simulink model "PDU"  (R2026b)
settings: Solver=VariableStepAuto
undefined symbols (not defined in the file or in its folder): P, Ts
libraries: nesl_utility x25, ee_lib x17, fl_lib x16, simulink x6, eeGeneralControl x3
settings Model: Creator=aomar  LastModifiedBy=aomar

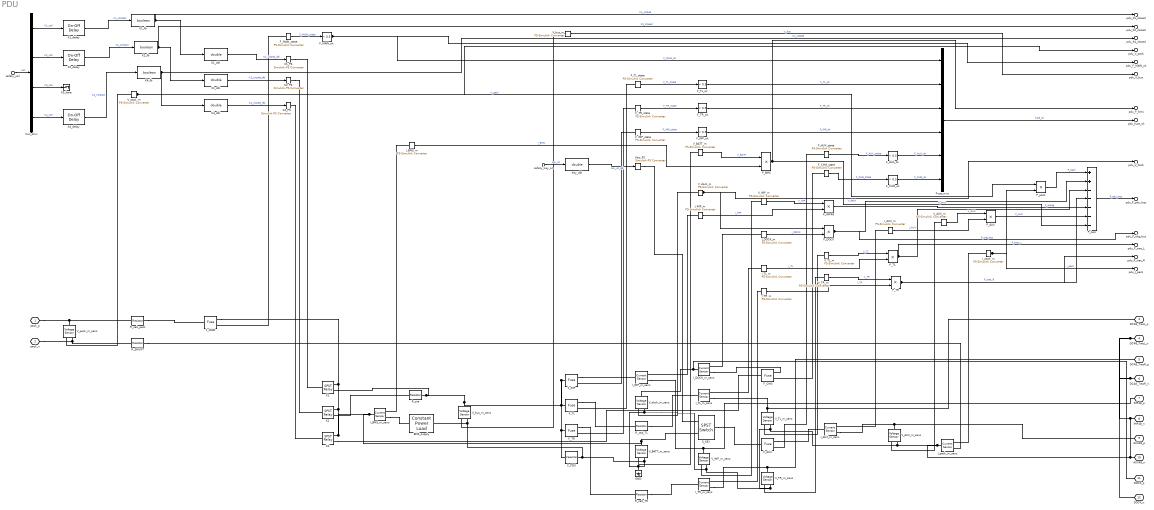
== system PDU ==
  safety_coil : Inport  PortName=safety  Element=coil
  safety_key_on : Inport  PortName=safety  Element=key_on
  BMS_supply : ee_lib/Passive/Constant Power Load  load_type=ee.enum.dc_ac.dc  consumed_power=P.power.pdu.P_bms_supply W  min_supply_voltage=20 V  G_reverse=1e-6 S  deltaV=1e-3 V  active_power=500 W  reactive_power=0 A*V  f0=60 Hz  Vrms_min=200 V  tau=0.01 s  Vrms_ini=300 V  Vang_ini=0 deg
  C_PDU : ee_lib/Passive/Capacitor  cap_option=ee.enum.passive.capacitor.capOption.const  c=P.power.pdu.C_pdu F  Cvec=[1e-05, 1e-06] F  Vvec=[0, 10] V  CV_table_symmetry=ee.enum.passive.capacitor.tableSymmetry.yes  f_vec=[1, 10] kHz  DFext_vec=[.8, 1.2]  enable_C_tol=ee.enum.toleranceApplication.none  averaging_period=0 s  C_tol=5  tol_distribution=ee.enum.toleranceDistribution.uniform  nSigma=4  r=P.power.pdu.ESR_pdu Ohm  g=P.power.pdu.g_bleed 1/Ohm  enable_operating_limits=ee.enum.enable.no  operating_limit_action=ee.enum.passive.reportOpLim.warn  max_working_voltage_range=[-25, 25] V  power_rating=1 W  maxTemperature=85 degC  thermalEnable=false  thermalMass=1 J/K  i_specify=off  i_priority=None  i=0 A  i_nominal_specify=off  i_nominal_value=1  i_nominal_unit=A  v_specify=off  v_priority=None  v=0 V  v_nominal_specify=off  v_nominal_value=1  v_nominal_unit=V  vc_specify=on  vc_priority=High  vc=0 V  vc_nominal_specify=off  vc_nominal_value=1  vc_nominal_unit=V  T_specify=off  T_priority=None  T=298.15 K  T_nominal_specify=off  T_nominal_value=1  T_nominal_unit=K
  Coil_dmx : Demux
  F_AUX : ee_lib/Switches & Breakers/Fuse  prm=3  I_rated=1 A  melt_margin=1  T_fuse=0 s  I2t=1 A^2*s  I_vec=P.power.pdu.F_AUX.I_vec A  t_vec=P.power.pdu.F_AUX.t_vec s  R_closed=P.power.pdu.F_AUX.R_closed Ohm  G_open=P.power.pdu.F_AUX.G_open 1/Ohm  exposemeasurement=ee.enum.exposemeasurement.visible
  F_AUX_ok : simulink/Logic and Bit Operations/Compare To Constant  relop=<  const=0.5  OutDataTypeStr=boolean
  F_AUX_state : nesl_utility/PS-Simulink Converter  PhysicalDomain=network_engine_domain  SubClassName=ps_output  LeftPortType=input  RightPortType=output  PseudoPeriodic=off  Frequencies=[]  VectorFormat=inherit  Unit=1  AffineConversion=off
  F_CHG : ee_lib/Switches & Breakers/Fuse  prm=3  I_rated=1 A  melt_margin=1  T_fuse=0 s  I2t=1 A^2*s  I_vec=P.power.pdu.F_CHG.I_vec A  t_vec=P.power.pdu.F_CHG.t_vec s  R_closed=P.power.pdu.F_CHG.R_closed Ohm  G_open=P.power.pdu.F_CHG.G_open 1/Ohm  exposemeasurement=ee.enum.exposemeasurement.visible
  F_CHG_ok : simulink/Logic and Bit Operations/Compare To Constant  relop=<  const=0.5  OutDataTypeStr=boolean
  F_CHG_state : nesl_utility/PS-Simulink Converter  PhysicalDomain=network_engine_domain  SubClassName=ps_output  LeftPortType=input  RightPortType=output  PseudoPeriodic=off  Frequencies=[]  VectorFormat=inherit  Unit=1  AffineConversion=off
  F_IMP : ee_lib/Switches & Breakers/Fuse  prm=3  I_rated=1 A  melt_margin=1  T_fuse=0 s  I2t=1 A^2*s  I_vec=P.power.pdu.F_IMP.I_vec A  t_vec=P.power.pdu.F_IMP.t_vec s  R_closed=P.power.pdu.F_IMP.R_closed Ohm  G_open=P.power.pdu.F_IMP.G_open 1/Ohm  exposemeasurement=ee.enum.exposemeasurement.visible
  F_IMP_ok : simulink/Logic and Bit Operations/Compare To Constant  relop=<  const=0.5  OutDataTypeStr=boolean
  F_IMP_state : nesl_utility/PS-Simulink Converter  PhysicalDomain=network_engine_domain  SubClassName=ps_output  LeftPortType=input  RightPortType=output  PseudoPeriodic=off  Frequencies=[]  VectorFormat=inherit  Unit=1  AffineConversion=off
  F_MAIN : ee_lib/Switches & Breakers/Fuse  prm=3  I_rated=1 A  melt_margin=1  T_fuse=0 s  I2t=1 A^2*s  I_vec=P.power.pdu.F_MAIN.I_vec A  t_vec=P.power.pdu.F_MAIN.t_vec s  R_closed=P.power.pdu.F_MAIN.R_closed Ohm  G_open=P.power.pdu.F_MAIN.G_open 1/Ohm  exposemeasurement=ee.enum.exposemeasurement.visible
  F_MAIN_ok : simulink/Logic and Bit Operations/Compare To Constant  relop=<  const=0.5  OutDataTypeStr=boolean
  F_MAIN_state : nesl_utility/PS-Simulink Converter  PhysicalDomain=network_engine_domain  SubClassName=ps_output  LeftPortType=input  RightPortType=output  PseudoPeriodic=off  Frequencies=[]  VectorFormat=inherit  Unit=1  AffineConversion=off
  F_TL : ee_lib/Switches & Breakers/Fuse  prm=3  I_rated=1 A  melt_margin=1  T_fuse=0 s  I2t=1 A^2*s  I_vec=P.power.pdu.F_TL.I_vec A  t_vec=P.power.pdu.F_TL.t_vec s  R_closed=P.power.pdu.F_TL.R_closed Ohm  G_open=P.power.pdu.F_TL.G_open 1/Ohm  exposemeasurement=ee.enum.exposemeasurement.visible
  F_TL_ok : simulink/Logic and Bit Operations/Compare To Constant  relop=<  const=0.5  OutDataTypeStr=boolean
  F_TL_state : nesl_utility/PS-Simulink Converter  PhysicalDomain=network_engine_domain  SubClassName=ps_output  LeftPortType=input  RightPortType=output  PseudoPeriodic=off  Frequencies=[]  VectorFormat=inherit  Unit=1  AffineConversion=off
  F_TR : ee_lib/Switches & Breakers/Fuse  prm=3  I_rated=1 A  melt_margin=1  T_fuse=0 s  I2t=1 A^2*s  I_vec=P.power.pdu.F_TR.I_vec A  t_vec=P.power.pdu.F_TR.t_vec s  R_closed=P.power.pdu.F_TR.R_closed Ohm  G_open=P.power.pdu.F_TR.G_open 1/Ohm  exposemeasurement=ee.enum.exposemeasurement.visible
  F_TR_ok : simulink/Logic and Bit Operations/Compare To Constant  relop=<  const=0.5  OutDataTypeStr=boolean
  F_TR_state : nesl_utility/PS-Simulink Converter  PhysicalDomain=network_engine_domain  SubClassName=ps_output  LeftPortType=input  RightPortType=output  PseudoPeriodic=off  Frequencies=[]  VectorFormat=inherit  Unit=1  AffineConversion=off
  Fuse_mux : Mux  Inputs=6
  GND : fl_lib/Electrical/Electrical Elements/Electrical Reference
  I_AUX_m : nesl_utility/PS-Simulink Converter  PhysicalDomain=network_engine_domain  SubClassName=ps_output  LeftPortType=input  RightPortType=output  PseudoPeriodic=off  Frequencies=[]  VectorFormat=inherit  Unit=A  AffineConversion=off
  I_AUX_m_sens : fl_lib/Electrical/Electrical Sensors/Current Sensor
  I_BMS_m : nesl_utility/PS-Simulink Converter  PhysicalDomain=network_engine_domain  SubClassName=ps_output  LeftPortType=input  RightPortType=output  PseudoPeriodic=off  Frequencies=[]  VectorFormat=inherit  Unit=A  AffineConversion=off
  I_BMS_m_sens : fl_lib/Electrical/Electrical Sensors/Current Sensor
  I_DOCK_m : nesl_utility/PS-Simulink Converter  PhysicalDomain=network_engine_domain  SubClassName=ps_output  LeftPortType=input  RightPortType=output  PseudoPeriodic=off  Frequencies=[]  VectorFormat=inherit  Unit=A  AffineConversion=off
  I_DOCK_m_sens : fl_lib/Electrical/Electrical Sensors/Current Sensor
  I_IMP_m : nesl_utility/PS-Simulink Converter  PhysicalDomain=network_engine_domain  SubClassName=ps_output  LeftPortType=input  RightPortType=output  PseudoPeriodic=off  Frequencies=[]  VectorFormat=inherit  Unit=A  AffineConversion=off
  I_IMP_m_sens : fl_lib/Electrical/Electrical Sensors/Current Sensor
  I_TL_m : nesl_utility/PS-Simulink Converter  PhysicalDomain=network_engine_domain  SubClassName=ps_output  LeftPortType=input  RightPortType=output  PseudoPeriodic=off  Frequencies=[]  VectorFormat=inherit  Unit=A  AffineConversion=off
  I_TL_m_sens : fl_lib/Electrical/Electrical Sensors/Current Sensor
  I_TR_m : nesl_utility/PS-Simulink Converter  PhysicalDomain=network_engine_domain  SubClassName=ps_output  LeftPortType=input  RightPortType=output  PseudoPeriodic=off  Frequencies=[]  VectorFormat=inherit  Unit=A  AffineConversion=off
  I_TR_m_sens : fl_lib/Electrical/Electrical Sensors/Current Sensor
  I_pack_m : nesl_utility/PS-Simulink Converter  PhysicalDomain=network_engine_domain  SubClassName=ps_output  LeftPortType=input  RightPortType=output  PseudoPeriodic=off  Frequencies=[]  VectorFormat=inherit  Unit=A  AffineConversion=off
  I_pack_m_sens : fl_lib/Electrical/Electrical Sensors/Current Sensor
  K1 : ee_lib/Switches & Breakers/Relays/SPST Relay  block_choices=ee.enum.controlport.ps  R_closed=P.power.pdu.K1.R_closed Ohm  G_open=P.power.pdu.K1.G_open 1/Ohm  Threshold=0.5  exposemeasurement=ee.enum.exposemeasurement.hidden  V_rated=5 V  V_energize=75  V_deenergize=25  l_winding=0.08 H  r_winding=12.5 Ohm  g_winding=1e-9 1/Ohm  T_brk_C_S=0 s  T_mak_C_S=0 s  fault_types=ee.enum.relays.faultTypes.winding
  K1_PS : nesl_utility/Simulink-PS Converter  PhysicalDomain=network_engine_domain  SubClassName=ps_input  LeftPortType=input  RightPortType=output  PseudoPeriodic=off  Frequencies=[]  NoiseDistribution=none  NoiseParameters=[]  Unit=1  AffineConversion=off  FilteringAndDerivatives=zero  SimscapeFilterOrder=1  InputFilterTimeConstant=0.001  UdotUserProvided=0
  K1_dbl : DataTypeConversion  OutDataTypeStr=double  SaturateOnIntegerOverflow=off  RndMeth=Floor
  K1_delay : eeGeneralControl/On-Off Delay  LabelModeActiveChoice=Discrete  Td_on=P.power.pdu.K1.t_on  Td_off=P.power.pdu.K1.t_off  IC=0  Ts=Ts.base
      settings: LibrarySourceBlock=ee_sl_lib/General Control/On-Off Delay
  K1_fb : DataTypeConversion  OutDataTypeStr=boolean  RndMeth=Nearest
  K2 : ee_lib/Switches & Breakers/Relays/SPST Relay  block_choices=ee.enum.controlport.ps  R_closed=P.power.pdu.K2.R_closed Ohm  G_open=P.power.pdu.K2.G_open 1/Ohm  Threshold=0.5  exposemeasurement=ee.enum.exposemeasurement.hidden  V_rated=5 V  V_energize=75  V_deenergize=25  l_winding=0.08 H  r_winding=12.5 Ohm  g_winding=1e-9 1/Ohm  T_brk_C_S=0 s  T_mak_C_S=0 s  fault_types=ee.enum.relays.faultTypes.winding
  K2_PS : nesl_utility/Simulink-PS Converter  PhysicalDomain=network_engine_domain  SubClassName=ps_input  LeftPortType=input  RightPortType=output  PseudoPeriodic=off  Frequencies=[]  NoiseDistribution=none  NoiseParameters=[]  Unit=1  AffineConversion=off  FilteringAndDerivatives=zero  SimscapeFilterOrder=1  InputFilterTimeConstant=0.001  UdotUserProvided=0
  K2_dbl : DataTypeConversion  OutDataTypeStr=double  SaturateOnIntegerOverflow=off  RndMeth=Floor
  K2_delay : eeGeneralControl/On-Off Delay  LabelModeActiveChoice=Discrete  Td_on=P.power.pdu.K2.t_on  Td_off=P.power.pdu.K2.t_off  IC=0  Ts=Ts.base
      settings: LibrarySourceBlock=ee_sl_lib/General Control/On-Off Delay
  K2_fb : DataTypeConversion  OutDataTypeStr=boolean  RndMeth=Nearest
  K3_here : Terminator
  K4 : ee_lib/Switches & Breakers/Relays/SPST Relay  block_choices=ee.enum.controlport.ps  R_closed=P.power.pdu.K4.R_closed Ohm  G_open=P.power.pdu.K4.G_open 1/Ohm  Threshold=0.5  exposemeasurement=ee.enum.exposemeasurement.hidden  V_rated=5 V  V_energize=75  V_deenergize=25  l_winding=0.08 H  r_winding=12.5 Ohm  g_winding=1e-9 1/Ohm  T_brk_C_S=0 s  T_mak_C_S=0 s  fault_types=ee.enum.relays.faultTypes.winding
  K4_PS : nesl_utility/Simulink-PS Converter  PhysicalDomain=network_engine_domain  SubClassName=ps_input  LeftPortType=input  RightPortType=output  PseudoPeriodic=off  Frequencies=[]  NoiseDistribution=none  NoiseParameters=[]  Unit=1  AffineConversion=off  FilteringAndDerivatives=zero  SimscapeFilterOrder=1  InputFilterTimeConstant=0.001  UdotUserProvided=0
  K4_dbl : DataTypeConversion  OutDataTypeStr=double  SaturateOnIntegerOverflow=off  RndMeth=Floor
  K4_delay : eeGeneralControl/On-Off Delay  LabelModeActiveChoice=Discrete  Td_on=P.power.pdu.K4.t_on  Td_off=P.power.pdu.K4.t_off  IC=0  Ts=Ts.base
      settings: LibrarySourceBlock=ee_sl_lib/General Control/On-Off Delay
  K4_fb : DataTypeConversion  OutDataTypeStr=boolean  RndMeth=Nearest
  Key_PS : nesl_utility/Simulink-PS Converter  PhysicalDomain=network_engine_domain  SubClassName=ps_input  LeftPortType=input  RightPortType=output  PseudoPeriodic=off  Frequencies=[]  NoiseDistribution=none  NoiseParameters=[]  Unit=V  AffineConversion=off  FilteringAndDerivatives=zero  SimscapeFilterOrder=1  InputFilterTimeConstant=0.001  UdotUserProvided=0
  Key_dbl : DataTypeConversion  OutDataTypeStr=double  SaturateOnIntegerOverflow=off  RndMeth=Floor
  P_AUX : Product
  P_BMS : Product
  P_DOCK : Product
  P_IMP48 : Product
  P_TL : Product
  P_TR : Product
  P_loss : Sum  Inputs=++-----
  P_pack : Product
  R_SHUNT : ee_lib/Passive/Resistor  R=P.power.pdu.R_shunt Ohm  enable_R_tol=ee.enum.toleranceApplication.none  R_tol=5  tol_distribution=ee.enum.toleranceDistribution.uniform  nSigma=4  enable_operating_limits=ee.enum.enable.no  operating_limit_action=ee.enum.passive.reportOpLim.warn  power_rating=1 W  max_working_voltage=100 V  noise_mode=ee.enum.sources.noise.Disabled  Tdevice=25 degC  sample_time=1e-3 s  repeatability=ee.enum.ic.repeatability.notRepeatable  user_seed=0  auto_seed=3254469079  power_derating_T1=70 degC  power_derating_T2=155 degC  operating_temperature_range_vec=[-50, 150] degC  alpha=3.93e-3 1/K  Tmeas=25 degC  thermal_mass=100 J/K  temperature_specify=off  temperature_priority=High  temperature=298.15 K  temperature_nominal_specify=off  temperature_nominal_value=1  temperature_nominal_unit=K
  R_cab_TL : ee_lib/Passive/Resistor  R=P.power.pdu.R_cab_trac Ohm  enable_R_tol=ee.enum.toleranceApplication.none  R_tol=5  tol_distribution=ee.enum.toleranceDistribution.uniform  nSigma=4  enable_operating_limits=ee.enum.enable.no  operating_limit_action=ee.enum.passive.reportOpLim.warn  power_rating=1 W  max_working_voltage=100 V  noise_mode=ee.enum.sources.noise.Disabled  Tdevice=25 degC  sample_time=1e-3 s  repeatability=ee.enum.ic.repeatability.notRepeatable  user_seed=0  auto_seed=4011470453  power_derating_T1=70 degC  power_derating_T2=155 degC  operating_temperature_range_vec=[-50, 150] degC  alpha=3.93e-3 1/K  Tmeas=25 degC  thermal_mass=100 J/K  temperature_specify=off  temperature_priority=High  temperature=298.15 K  temperature_nominal_specify=off  temperature_nominal_value=1  temperature_nominal_unit=K
  R_cab_TR : ee_lib/Passive/Resistor  R=P.power.pdu.R_cab_trac Ohm  enable_R_tol=ee.enum.toleranceApplication.none  R_tol=5  tol_distribution=ee.enum.toleranceDistribution.uniform  nSigma=4  enable_operating_limits=ee.enum.enable.no  operating_limit_action=ee.enum.passive.reportOpLim.warn  power_rating=1 W  max_working_voltage=100 V  noise_mode=ee.enum.sources.noise.Disabled  Tdevice=25 degC  sample_time=1e-3 s  repeatability=ee.enum.ic.repeatability.notRepeatable  user_seed=0  auto_seed=2915145293  power_derating_T1=70 degC  power_derating_T2=155 degC  operating_temperature_range_vec=[-50, 150] degC  alpha=3.93e-3 1/K  Tmeas=25 degC  thermal_mass=100 J/K  temperature_specify=off  temperature_priority=High  temperature=298.15 K  temperature_nominal_specify=off  temperature_nominal_value=1  temperature_nominal_unit=K
  R_cab_pack : ee_lib/Passive/Resistor  R=P.power.pdu.R_cab_pack Ohm  enable_R_tol=ee.enum.toleranceApplication.none  R_tol=5  tol_distribution=ee.enum.toleranceDistribution.uniform  nSigma=4  enable_operating_limits=ee.enum.enable.no  operating_limit_action=ee.enum.passive.reportOpLim.warn  power_rating=1 W  max_working_voltage=100 V  noise_mode=ee.enum.sources.noise.Disabled  Tdevice=25 degC  sample_time=1e-3 s  repeatability=ee.enum.ic.repeatability.notRepeatable  user_seed=0  auto_seed=153380492  power_derating_T1=70 degC  power_derating_T2=155 degC  operating_temperature_range_vec=[-50, 150] degC  alpha=3.93e-3 1/K  Tmeas=25 degC  thermal_mass=100 J/K  temperature_specify=off  temperature_priority=High  temperature=298.15 K  temperature_nominal_specify=off  temperature_nominal_value=1  temperature_nominal_unit=K
  R_pre : ee_lib/Passive/Resistor  R=P.power.pdu.R_pre Ohm  enable_R_tol=ee.enum.toleranceApplication.none  R_tol=5  tol_distribution=ee.enum.toleranceDistribution.uniform  nSigma=4  enable_operating_limits=ee.enum.enable.no  operating_limit_action=ee.enum.passive.reportOpLim.warn  power_rating=1 W  max_working_voltage=100 V  noise_mode=ee.enum.sources.noise.Disabled  Tdevice=25 degC  sample_time=1e-3 s  repeatability=ee.enum.ic.repeatability.notRepeatable  user_seed=0  auto_seed=3646982598  power_derating_T1=70 degC  power_derating_T2=155 degC  operating_temperature_range_vec=[-50, 150] degC  alpha=3.93e-3 1/K  Tmeas=25 degC  thermal_mass=100 J/K  temperature_specify=off  temperature_priority=High  temperature=298.15 K  temperature_nominal_specify=off  temperature_nominal_value=1  temperature_nominal_unit=K
  S_KEY : ee_lib/Switches & Breakers/SPST Switch  R_closed=P.power.pdu.R_key Ohm  G_open=1e-8 S  Threshold=0.5 V  Width=0 V  model_dynamics=0  t_on=1e-3 s  t_off=1e-3 s  initial_vT=0 V
  V_AUX_m : nesl_utility/PS-Simulink Converter  PhysicalDomain=network_engine_domain  SubClassName=ps_output  LeftPortType=input  RightPortType=output  PseudoPeriodic=off  Frequencies=[]  VectorFormat=inherit  Unit=V  AffineConversion=off
  V_AUX_m_sens : fl_lib/Electrical/Electrical Sensors/Voltage Sensor
  V_BATT_m : nesl_utility/PS-Simulink Converter  PhysicalDomain=network_engine_domain  SubClassName=ps_output  LeftPortType=input  RightPortType=output  PseudoPeriodic=off  Frequencies=[]  VectorFormat=inherit  Unit=V  AffineConversion=off
  V_BATT_m_sens : fl_lib/Electrical/Electrical Sensors/Voltage Sensor
  V_IMP_m : nesl_utility/PS-Simulink Converter  PhysicalDomain=network_engine_domain  SubClassName=ps_output  LeftPortType=input  RightPortType=output  PseudoPeriodic=off  Frequencies=[]  VectorFormat=inherit  Unit=V  AffineConversion=off
  V_IMP_m_sens : fl_lib/Electrical/Electrical Sensors/Voltage Sensor
  V_TL_m : nesl_utility/PS-Simulink Converter  PhysicalDomain=network_engine_domain  SubClassName=ps_output  LeftPortType=input  RightPortType=output  PseudoPeriodic=off  Frequencies=[]  VectorFormat=inherit  Unit=V  AffineConversion=off
  V_TL_m_sens : fl_lib/Electrical/Electrical Sensors/Voltage Sensor
  V_TR_m : nesl_utility/PS-Simulink Converter  PhysicalDomain=network_engine_domain  SubClassName=ps_output  LeftPortType=input  RightPortType=output  PseudoPeriodic=off  Frequencies=[]  VectorFormat=inherit  Unit=V  AffineConversion=off
  V_TR_m_sens : fl_lib/Electrical/Electrical Sensors/Voltage Sensor
  V_bus_m : nesl_utility/PS-Simulink Converter  PhysicalDomain=network_engine_domain  SubClassName=ps_output  LeftPortType=input  RightPortType=output  PseudoPeriodic=off  Frequencies=[]  VectorFormat=inherit  Unit=V  AffineConversion=off
  V_bus_m_sens : fl_lib/Electrical/Electrical Sensors/Voltage Sensor
  V_dock_m : nesl_utility/PS-Simulink Converter  PhysicalDomain=network_engine_domain  SubClassName=ps_output  LeftPortType=input  RightPortType=output  PseudoPeriodic=off  Frequencies=[]  VectorFormat=inherit  Unit=V  AffineConversion=off
  V_dock_m_sens : fl_lib/Electrical/Electrical Sensors/Voltage Sensor
  V_pack_m : nesl_utility/PS-Simulink Converter  PhysicalDomain=network_engine_domain  SubClassName=ps_output  LeftPortType=input  RightPortType=output  PseudoPeriodic=off  Frequencies=[]  VectorFormat=inherit  Unit=V  AffineConversion=off
  V_pack_m_sens : fl_lib/Electrical/Electrical Sensors/Voltage Sensor
  pack_p : PMIOPort  Side=Left  ConnectionType=Connection: foundation.electrical.electrical
  pack_n : PMIOPort  Port=2  Side=Left  ConnectionType=Connection: foundation.electrical.electrical
  DC48_TracL_p : PMIOPort  Port=3  Side=Right  ConnectionType=Connection: foundation.electrical.electrical
  DC48_TracL_n : PMIOPort  Port=4  Side=Right  ConnectionType=Connection: foundation.electrical.electrical
  DC48_TracR_p : PMIOPort  Port=5  Side=Right  ConnectionType=Connection: foundation.electrical.electrical
  DC48_TracR_n : PMIOPort  Port=6  Side=Right  ConnectionType=Connection: foundation.electrical.electrical
  IMP48_p : PMIOPort  Port=7  Side=Right  ConnectionType=Connection: foundation.electrical.electrical
  IMP48_n : PMIOPort  Port=8  Side=Right  ConnectionType=Connection: foundation.electrical.electrical
  AUX48_p : PMIOPort  Port=9  Side=Right  ConnectionType=Connection: foundation.electrical.electrical
  AUX48_n : PMIOPort  Port=10  Side=Right  ConnectionType=Connection: foundation.electrical.electrical
  DOCK_p : PMIOPort  Port=11  Side=Right  ConnectionType=Connection: foundation.electrical.electrical
  DOCK_n : PMIOPort  Port=12  Side=Right  ConnectionType=Connection: foundation.electrical.electrical
  pdu_V_pack : Outport  PortName=pdu  Element=V_pack
  pdu_V_bus : Outport  PortName=pdu  Element=V_bus
  pdu_V_dock : Outport  PortName=pdu  Element=V_dock
  pdu_I_pack : Outport  PortName=pdu  Element=I_pack
  pdu_K1_closed : Outport  PortName=pdu  Element=K1_closed
  pdu_K2_closed : Outport  PortName=pdu  Element=K2_closed
  pdu_K4_closed : Outport  PortName=pdu  Element=K4_closed
  pdu_fuse_ok : Outport  PortName=pdu  Element=fuse_ok
  pdu_F_MAIN_ok : Outport  PortName=pdu  Element=F_MAIN_ok
  pdu_P_trac_L : Outport  PortName=pdu  Element=P_trac_L
  pdu_P_trac_R : Outport  PortName=pdu  Element=P_trac_R
  pdu_P_chg_bus : Outport  PortName=pdu  Element=P_chg_bus
  pdu_P_pdu_loss : Outport  PortName=pdu  Element=P_pdu_loss
  pdu_P_bms : Outport  PortName=pdu  Element=P_bms
  wires:
  safety_coil/1 -> Coil_dmx/1  "coil"
  Coil_dmx/1 -> K1_delay/1  "K1_coil"
  Coil_dmx/2 -> K2_delay/1  "K2_coil"
  Coil_dmx/3 -> K3_here/1  "K3_coil"
  Coil_dmx/4 -> K4_delay/1  "K4_coil"
  K1_delay/1 -> K1_fb/1  "K1_contact"
  K2_delay/1 -> K2_fb/1  "K2_contact"
  K4_delay/1 -> K4_fb/1  "K4_contact"
  V_pack_m/1 -> P_pack/1, pdu_V_pack/1  "V_pack"
  K1_fb/1 -> K1_dbl/1, pdu_K1_closed/1  "K1_closed"
  K2_fb/1 -> K2_dbl/1, pdu_K2_closed/1  "K2_closed"
  K4_fb/1 -> pdu_K4_closed/1, K4_dbl/1  "K4_closed"
  K1_dbl/1 -> K1_PS/1  "K1_closed_dbl"
  K2_dbl/1 -> K2_PS/1  "K2_closed_dbl"
  K4_dbl/1 -> K4_PS/1  "K4_closed_dbl"
  F_MAIN_state/1 -> F_MAIN_ok/1  "F_MAIN_state"
  F_MAIN_ok/1 -> pdu_F_MAIN_ok/1, Fuse_mux/1  "F_MAIN_ok"
  I_BMS_m/1 -> P_BMS/2  "I_BMS"
  safety_key_on/1 -> Key_dbl/1  "key_on"
  V_bus_m/1 -> pdu_V_bus/1  "V_bus"
  Key_dbl/1 -> Key_PS/1  "key_on_dbl"
  F_TL_state/1 -> F_TL_ok/1  "F_TL_state"
  F_TR_state/1 -> F_TR_ok/1  "F_TR_state"
  F_IMP_state/1 -> F_IMP_ok/1  "F_IMP_state"
  V_BATT_m/1 -> P_BMS/1  "V_BATT"
  V_dock_m/1 -> P_DOCK/1, pdu_V_dock/1  "V_dock"
  I_IMP_m/1 -> P_IMP48/2  "I_IMP"
  F_TL_ok/1 -> Fuse_mux/2  "F_TL_ok"
  F_TR_ok/1 -> Fuse_mux/3  "F_TR_ok"
  F_IMP_ok/1 -> Fuse_mux/4  "F_IMP_ok"
  V_IMP_m/1 -> P_IMP48/1  "V_IMP"
  I_DOCK_m/1 -> P_DOCK/2  "I_DOCK"
  I_TL_m/1 -> P_TL/2  "I_TL"
  I_TR_m/1 -> P_TR/2  "I_TR"
  P_BMS/1 -> P_loss/7, pdu_P_bms/1  "P_bms"
  F_AUX_state/1 -> F_AUX_ok/1  "F_AUX_state"
  F_CHG_state/1 -> F_CHG_ok/1  "F_CHG_state"
  V_TL_m/1 -> P_TL/1  "V_TL"
  V_TR_m/1 -> P_TR/1  "V_TR"
  P_IMP48/1 -> P_loss/5  "P_IMP48"
  P_DOCK/1 -> P_loss/2, pdu_P_chg_bus/1  "P_chg_bus"
  I_AUX_m/1 -> P_AUX/2  "I_AUX"
  F_AUX_ok/1 -> Fuse_mux/5  "F_AUX_ok"
  F_CHG_ok/1 -> Fuse_mux/6  "F_CHG_ok"
  P_TL/1 -> P_loss/3, pdu_P_trac_L/1  "P_trac_L"
  P_TR/1 -> P_loss/4, pdu_P_trac_R/1  "P_trac_R"
  Fuse_mux/1 -> pdu_fuse_ok/1  "fuse_ok"
  V_AUX_m/1 -> P_AUX/1  "V_AUX"
  I_pack_m/1 -> P_pack/2, pdu_I_pack/1  "I_pack"
  P_AUX/1 -> P_loss/6  "P_AUX"
  P_pack/1 -> P_loss/1  "P_pack"
  P_loss/1 -> pdu_P_pdu_loss/1  "P_pdu_loss"
  connections:
  V_AUX_m_sens/LConn1 -- I_AUX_m_sens/RConn2 -- AUX48_p/RConn1
  I_BMS_m_sens/RConn2 -- BMS_supply/LConn1
  R_pre/RConn1 -- K1/RConn2 -- V_bus_m_sens/LConn1 -- F_TL/LConn1 -- F_IMP/LConn1 -- F_TR/LConn1 -- C_PDU/LConn1
  V_TL_m_sens/LConn1 -- I_TL_m_sens/RConn2 -- DC48_TracL_p/RConn1
  V_TR_m_sens/LConn1 -- I_TR_m_sens/RConn2 -- DC48_TracR_p/RConn1
  I_DOCK_m_sens/LConn1 -- V_dock_m_sens/LConn1 -- DOCK_p/RConn1
  S_KEY/RConn1 -- F_AUX/LConn1
  F_AUX/RConn1 -- I_AUX_m_sens/LConn1
  F_AUX_state/LConn1 -- F_AUX/RConn2
  K4/RConn2 -- F_CHG/LConn1
  I_DOCK_m_sens/RConn2 -- F_CHG/RConn1
  F_CHG_state/LConn1 -- F_CHG/RConn2
  F_IMP/RConn1 -- I_IMP_m_sens/LConn1
  F_IMP_state/LConn1 -- F_IMP/RConn2
  R_cab_pack/RConn1 -- F_MAIN/LConn1
  K1/RConn1 -- F_MAIN/RConn1 -- K2/RConn1 -- K4/RConn1 -- I_BMS_m_sens/LConn1 -- V_BATT_m_sens/LConn1 -- S_KEY/LConn2
  F_MAIN_state/LConn1 -- F_MAIN/RConn2
  F_TL/RConn1 -- R_cab_TL/LConn1
  F_TL_state/LConn1 -- F_TL/RConn2
  F_TR/RConn1 -- R_cab_TR/LConn1
  F_TR_state/LConn1 -- F_TR/RConn2
  V_IMP_m_sens/LConn1 -- I_IMP_m_sens/RConn2 -- IMP48_p/RConn1
  I_AUX_m/LConn1 -- I_AUX_m_sens/RConn1
  I_BMS_m/LConn1 -- I_BMS_m_sens/RConn1
  I_DOCK_m/LConn1 -- I_DOCK_m_sens/RConn1
  I_IMP_m/LConn1 -- I_IMP_m_sens/RConn1
  I_TL_m/LConn1 -- I_TL_m_sens/RConn1
  R_cab_TL/RConn1 -- I_TL_m_sens/LConn1
  I_TR_m/LConn1 -- I_TR_m_sens/RConn1
  R_cab_TR/RConn1 -- I_TR_m_sens/LConn1
  I_pack_m/LConn1 -- I_pack_m_sens/RConn1
  R_SHUNT/RConn1 -- I_pack_m_sens/RConn2
  K1_PS/RConn1 -- K1/LConn1
  K2_PS/RConn1 -- K2/LConn1
  K2/RConn2 -- R_pre/LConn1
  K4_PS/RConn1 -- K4/LConn1
  Key_PS/RConn1 -- S_KEY/LConn1
  V_pack_m_sens/RConn2 -- pack_n/RConn1 -- R_SHUNT/LConn1
  V_pack_m_sens/LConn1 -- pack_p/RConn1 -- R_cab_pack/LConn1
  V_AUX_m/LConn1 -- V_AUX_m_sens/RConn1
  V_IMP_m/LConn1 -- V_IMP_m_sens/RConn1
  V_TL_m/LConn1 -- V_TL_m_sens/RConn1
  V_TR_m/LConn1 -- V_TR_m_sens/RConn1
  V_bus_m/LConn1 -- V_bus_m_sens/RConn1
  V_dock_m/LConn1 -- V_dock_m_sens/RConn1
  V_pack_m/LConn1 -- V_pack_m_sens/RConn1
  DC48_TracL_n/RConn1 -- DOCK_n/RConn1 -- DC48_TracR_n/RConn1 -- IMP48_n/RConn1 -- AUX48_n/RConn1 -- I_pack_m_sens/LConn1 -- V_AUX_m_sens/RConn2 -- V_TL_m_sens/RConn2 -- V_TR_m_sens/RConn2 -- V_IMP_m_sens/RConn2 -- V_dock_m_sens/RConn2 -- GND/LConn1 -- V_BATT_m_sens/RConn2 -- C_PDU/RConn1 -- V_bus_m_sens/RConn2 -- BMS_supply/RConn1
  V_BATT_m/LConn1 -- V_BATT_m_sens/RConn1
